simulink model "flexible_shaft_ctrl"  (R2025b)
settings: Solver=ode1be  StartTime=0.0  StopTime=simlength  FixedStep=tc  RelTol=1e-3  EnableMultiTasking=on
values from neighbouring files (symbols this model uses):
  Aled = eye(4) + Ale*ts_slow    [init.m]
  Bled = Ble*ts_slow    [init.m]
  Cle = [1 0 0 0]    [init.m]
  Dl = torque_nom/5    (= 64800)    [model1_parameters.m]    (also in model2_parameters.m = 39000; model_parameters_derivation.m = 18000)
  Dm = torque_nom/5    (= 64800)    [model1_parameters.m]    (also in model2_parameters.m = 39000; model_parameters_derivation.m = 18000)
  Dtheta = torque_nom/50    (= 6480)    [model1_parameters.m]    (also in model2_parameters.m = 3900; model_parameters_derivation.m = 18000)
  f0_min = 1/2/pi*sqrt(Ktheta*(1/Jm_max+1/Jl_max))    [model1_parameters.m]    (also in model2_parameters.m; model_parameters_derivation.m)
  Jl_model = Jl_max    [init.m]
  Jm_model = Jm_max    [init.m]
  ki = 12.5    [init.m]
  kp = 2    [init.m]
  Ksf = [0, 0, 0, 0]    [init.m]
  Lle = (lqr(Ale',Cle',Qle,Rle))'    [init.m]
  omega_nom = omega_nom_rpm/60*2*pi    (= 2.85714285714)    [model1_parameters.m]    (also in model2_parameters.m = 2.44897959184)
  omega_ref_pu = 1    [init.m]
  slope_down = 1    [init.m]
  slope_rise = 1    [init.m]
  stop = 50    [init.m]
  tc = ts_fast/2    (= 8.06451612903e-05)    [init.m]
  time_start = 0.1    [init.m]
  torque_disturbance = 0.1    [init.m]
  torque_m_pu_lim = 1.4    [init.m]
  torque_nom = 324e3    (= 324000)    [model1_parameters.m]    (also in model2_parameters.m = 195000; model_parameters_derivation.m = 180000)
  ts_fast = 1/fPWM/2    (= 0.000161290322581)    [init.m]
  ts_slow = ts_fast*SYS_TIMEBASE_FACTOR    (= 0.00129032258065)    [init.m]
  young_module_rope = 100.75e3    (= 100750)    [model1_parameters.m]    (also in model2_parameters.m; model_parameters_derivation.m = 125000)
libraries: nesl_utility x12, fl_lib x10, flexshaft_2masses_lib x2, cstblocks x1
settings Model: SimulationMode=accelerator  Creator=ltnbda  LastModifiedBy=dbagn
settings SolverCC: AlgebraicLoopSolver=TrustRegion  AutoInsertRateTranBlk=on
settings DataIOCC: LimitDataPoints=on  SaveFormat=Array  SaveOutput=off  SignalLogging=off  DSMLogging=off  SaveTime=off  ReturnWorkspaceOutputs=off
settings OptimizationCC: ReuseModelBlockBuffer=off  ExpressionDepthLimit=2147483647.0  LifeSpan=inf
settings DebuggingCC: UnderspecifiedInitializationDetection=Classic  MergeDetectMultiDrivingBlocksExec=none  SolverPrmCheckMsg=warning  UnconnectedInputMsg=warning  UnconnectedOutputMsg=warning  UnconnectedLineMsg=warning  StateNameClashWarn=warning  SFUnexpectedBacktrackingDiag=warning  SFNoUnconditionalDefaultTransitionDiag=warning  SFExecutionAtInitializationDiag=none  ArithmeticOperatorsInVariantConditions=warning
settings HardwareCC: ProdBitPerPointer=32.0  ProdBitPerSizeT=32.0  ProdBitPerPtrDiffT=32.0  ProdLargestAtomicFloat=None  ProdIntDivRoundTo=Undefined  ProdEndianess=Unspecified  ProdWordSize=32.0  ProdHWDeviceType=32-bit Generic
settings ModelReferenceCC: EnableRefExpFcnMdlSchedulingChecks=on  PropagateSignalLabelsOutOfModel=off
settings SFSimCC: SimUseLocalCustomCode=off  CustomCodeUndefinedFunction=UseInterfaceOnly
settings SFSimCC: SimCustomHeaderCode=|
  | #include "advanced_speed_control.h"
  | #include "advanced_speed_control_simulink.h"
  | #include "adv_speed_ctrl_pisf.h"
  | #include "adv_speed_ctrl_pisf_simulink.h"
  | #include "adv_speed_ctrl_pisfle.h"
  | #include "adv_speed_ctrl_pisfle_simulink.h"
settings SFSimCC: SimUserSources=|
  | "advanced_speed_control_simulink.c"
  | "advanced_speed_control.c"
  | "adv_speed_ctrl_pisf_simulink.c"
  | "adv_speed_ctrl_pisf.c"
  | "adv_speed_ctrl_pisfle_simulink.c"
  | "adv_speed_ctrl_pisfle.c"
settings SFSimCC: SimUserIncludeDirs=|
  | include
  | src
settings RTWCC: RTWUseLocalCustomCode=off  GPUComputeCapability=3.5
settings CodeAppCC: StateflowObjectComments=on
settings GRTTargetCC: TargetLangStandard=C89/C90 (ANSI)
settings ConfigComp: CovMetricSettings=dw  CovSaveCumulativeToWorkspaceVar=on  CovSaveSingleToWorkspaceVar=on  CovExternalEMLEnable=off

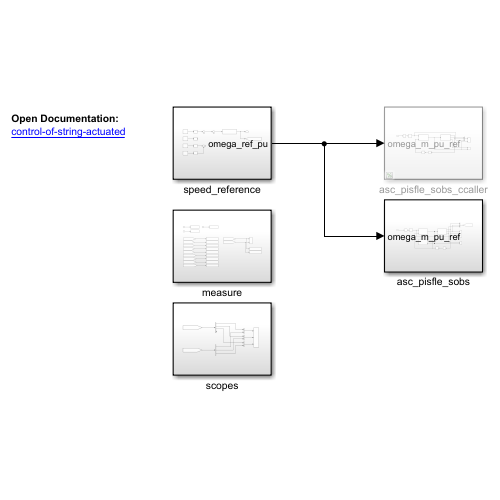
[thumbnail: Simulink's stored preview of the top-level diagram]
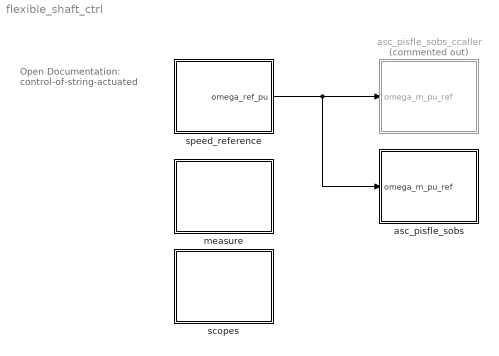
== system flexible_shaft_ctrl ==
  note: Open Documentation:
      | control-of-string-actuated
  asc_pisfle_sobs : Subsystem
  asc_pisfle_sobs_ccaller : Subsystem  Commented=on
  measure : Subsystem
  scopes : Subsystem
  speed_reference : Subsystem
  wires:
  speed_reference/1(omega_ref_pu) -> asc_pisfle_sobs_ccaller/1(omega_m_pu_ref), asc_pisfle_sobs/1(omega_m_pu_ref)

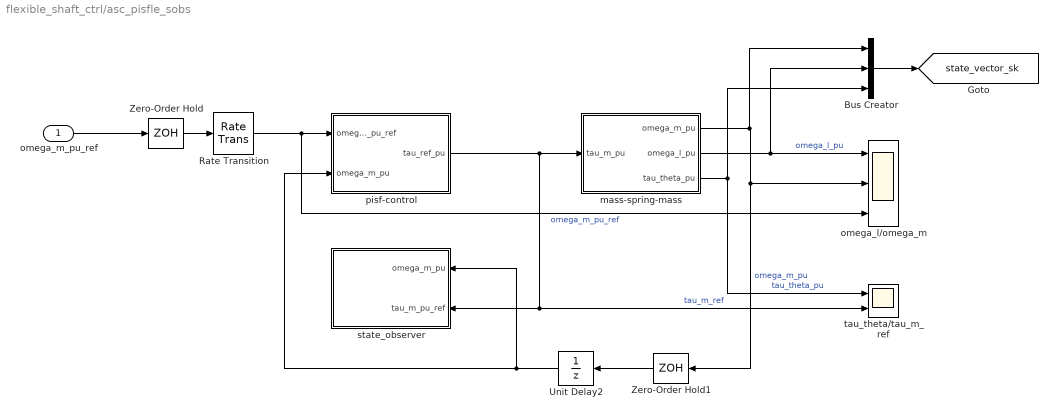
== system flexible_shaft_ctrl/asc_pisfle_sobs ==
  omega_m_pu_ref : Inport
  Bus Creator : BusCreator  Inputs=3
  Rate Transition : RateTransition  OutPortSampleTime=ts_slow
  Unit Delay2 : UnitDelay  SampleTime=ts_slow  HasFrameUpgradeWarning=on
  Zero-Order Hold : ZeroOrderHold  SampleTime=ts_slow
  Zero-Order Hold1 : ZeroOrderHold  SampleTime=ts_slow
  mass-spring-mass : Subsystem
  omega_l/omega_m : Scope  NumInputPorts=3
      settings: ActiveDisplayYMinimum=-0.17271134973649729  ActiveDisplayYMaximum=1.5544021476284759
  pisf-control : Subsystem
  state_observer : Subsystem
  tau_theta/tau_m_ref : Scope  NumInputPorts=2
      settings: ActiveDisplayYMinimum=-1.2903878055625353  ActiveDisplayYMaximum=1.6989319783958372
  tag scope: state_vector_sk=global
  wires:
  Unit Delay2/1 -> state_observer/1(omega_m_pu), pisf-control/2(omega_m_pu)
  mass-spring-mass/2(omega_l_pu) -> Bus Creator/2, omega_l/omega_m/1  "omega_l_pu"
  Zero-Order Hold1/1 -> Unit Delay2/1
  mass-spring-mass/1(omega_m_pu) -> Bus Creator/1, Zero-Order Hold1/1, omega_l/omega_m/2  "omega_m_pu"
  mass-spring-mass/3(tau_theta_pu) -> Bus Creator/3, tau_theta/tau_m_ref/1  "tau_theta_pu"
  omega_m_pu_ref/1 -> Zero-Order Hold/1
  Rate Transition/1 -> pisf-control/1(omega_m_pu_ref), omega_l/omega_m/3  "omega_m_pu_ref"
  pisf-control/1(tau_ref_pu) -> state_observer/2(tau_m_pu_ref), tau_theta/tau_m_ref/2, mass-spring-mass/1(tau_m_pu)  "tau_m_ref"
  Zero-Order Hold/1 -> Rate Transition/1
  Bus Creator/1 -> [state_vector_sk]

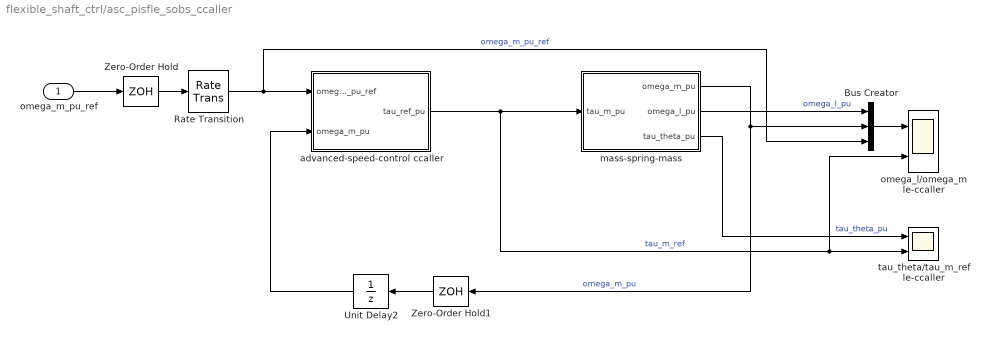
== system flexible_shaft_ctrl/asc_pisfle_sobs_ccaller ==
  omega_m_pu_ref : Inport
  Bus Creator : BusCreator  Inputs=3
  Rate Transition : RateTransition  OutPortSampleTime=ts_slow
  Unit Delay2 : UnitDelay  SampleTime=ts_slow  HasFrameUpgradeWarning=on
  Zero-Order Hold : ZeroOrderHold  SampleTime=ts_slow
  Zero-Order Hold1 : ZeroOrderHold  SampleTime=ts_slow
  advanced-speed-control ccaller : Subsystem
  mass-spring-mass : Subsystem
  omega_l/omega_m le-ccaller : Scope  NumInputPorts=2
      settings: SampleTime=ts_slow  ActiveDisplayYMinimum=-0.2317  ActiveDisplayYMaximum=2.0853
  tau_theta/tau_m_ref le-ccaller : Scope  NumInputPorts=2
      settings: SampleTime=tc  ActiveDisplayYMinimum=-0.175  ActiveDisplayYMaximum=1.575
  wires:
  Unit Delay2/1 -> advanced-speed-control ccaller/2(omega_m_pu)
  mass-spring-mass/2(omega_l_pu) -> Bus Creator/1  "omega_l_pu"
  Zero-Order Hold1/1 -> Unit Delay2/1
  mass-spring-mass/1(omega_m_pu) -> Bus Creator/2, Zero-Order Hold1/1  "omega_m_pu"
  mass-spring-mass/3(tau_theta_pu) -> tau_theta/tau_m_ref le-ccaller/1  "tau_theta_pu"
  omega_m_pu_ref/1 -> Zero-Order Hold/1
  Zero-Order Hold/1 -> Rate Transition/1
  advanced-speed-control ccaller/1(tau_ref_pu) -> omega_l/omega_m le-ccaller/2, tau_theta/tau_m_ref le-ccaller/2, mass-spring-mass/1(tau_m_pu)  "tau_m_ref"
  Bus Creator/1 -> omega_l/omega_m le-ccaller/1
  Rate Transition/1 -> Bus Creator/3, advanced-speed-control ccaller/1(omega_m_pu_ref)  "omega_m_pu_ref"

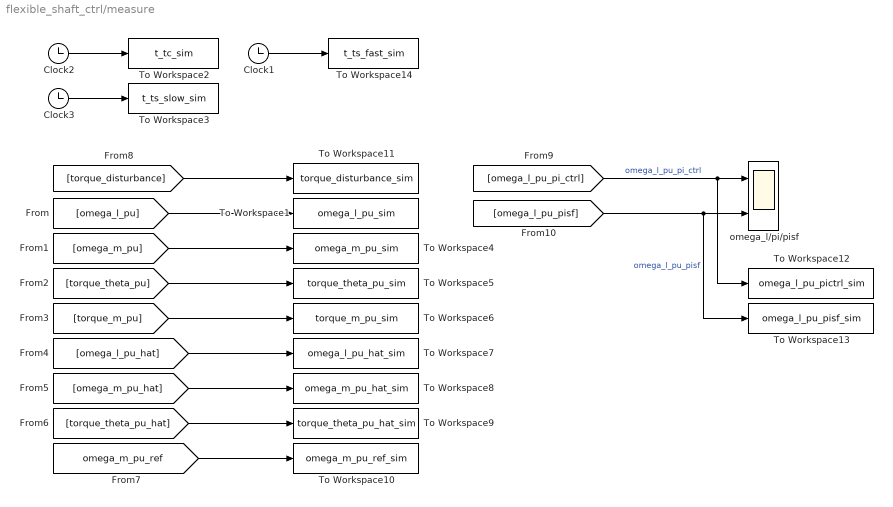
== system flexible_shaft_ctrl/measure ==
  Clock1 : Clock
  Clock2 : Clock
  Clock3 : Clock
  To Workspace1 : ToWorkspace  VariableName=omega_l_pu_sim  SampleTime=tc
      settings: MaxDataPoints=Nc
  To Workspace10 : ToWorkspace  VariableName=omega_m_pu_ref_sim  SampleTime=tc
      settings: MaxDataPoints=Nc
  To Workspace11 : ToWorkspace  VariableName=torque_disturbance_sim  SampleTime=tc
      settings: MaxDataPoints=Nc
  To Workspace12 : ToWorkspace  VariableName=omega_l_pu_pictrl_sim  SampleTime=tc
      settings: MaxDataPoints=Nc
  To Workspace13 : ToWorkspace  VariableName=omega_l_pu_pisf_sim  SampleTime=tc
      settings: MaxDataPoints=Nc
  To Workspace14 : ToWorkspace  VariableName=t_ts_fast_sim  SampleTime=ts_fast
      settings: MaxDataPoints=Ns_fast
  To Workspace2 : ToWorkspace  VariableName=t_tc_sim  SampleTime=tc
      settings: MaxDataPoints=Nc
  To Workspace3 : ToWorkspace  VariableName=t_ts_slow_sim  SampleTime=ts_slow
      settings: MaxDataPoints=Ns_slow
  To Workspace4 : ToWorkspace  VariableName=omega_m_pu_sim  SampleTime=tc
      settings: MaxDataPoints=Nc
  To Workspace5 : ToWorkspace  VariableName=torque_theta_pu_sim  SampleTime=tc
      settings: MaxDataPoints=Nc
  To Workspace6 : ToWorkspace  VariableName=torque_m_pu_sim  SampleTime=tc
      settings: MaxDataPoints=Nc
  To Workspace7 : ToWorkspace  VariableName=omega_l_pu_hat_sim  SampleTime=tc
      settings: MaxDataPoints=Nc
  To Workspace8 : ToWorkspace  VariableName=omega_m_pu_hat_sim  SampleTime=tc
      settings: MaxDataPoints=Nc
  To Workspace9 : ToWorkspace  VariableName=torque_theta_pu_hat_sim  SampleTime=tc
      settings: MaxDataPoints=Nc
  omega_l/pi/pisf : Scope  NumInputPorts=2
      settings: SampleTime=tc  ActiveDisplayYMinimum=-0.18711  ActiveDisplayYMaximum=1.68397
  wires:
  Clock2/1 -> To Workspace2/1
  Clock3/1 -> To Workspace3/1
  [omega_l_pu] -> To Workspace1/1
  [omega_m_pu] -> To Workspace4/1
  [torque_theta_pu] -> To Workspace5/1
  [torque_m_pu] -> To Workspace6/1
  [omega_l_pu_hat] -> To Workspace7/1
  [omega_m_pu_hat] -> To Workspace8/1
  [torque_theta_pu_hat] -> To Workspace9/1
  [omega_m_pu_ref] -> To Workspace10/1
  [torque_disturbance] -> To Workspace11/1
  [omega_l_pu_pisf] -> To Workspace13/1, omega_l/pi/pisf/2  "omega_l_pu_pisf"
  [omega_l_pu_pi_ctrl] -> To Workspace12/1, omega_l/pi/pisf/1  "omega_l_pu_pi_ctrl"
  Clock1/1 -> To Workspace14/1

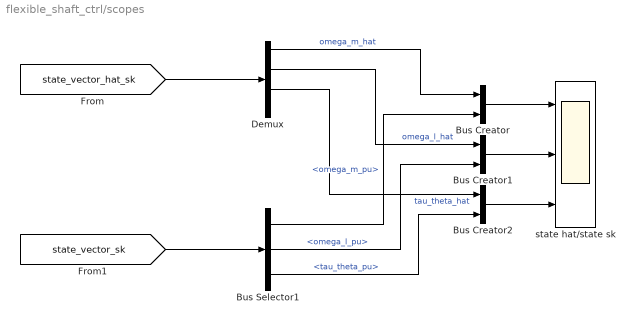
== system flexible_shaft_ctrl/scopes ==
  Bus Creator : BusCreator  Inputs=2
  Bus Creator1 : BusCreator  Inputs=2
  Bus Creator2 : BusCreator  Inputs=2
  Bus Selector1 : BusSelector  OutputSignals=omega_m_pu,omega_l_pu,tau_theta_pu
  Demux : Demux
  state hat/state sk : Scope  NumInputPorts=3
      settings: ActiveDisplayString=3  ActiveDisplayYMinimum=-0.14809096846427292  ActiveDisplayYMaximum=1.3328187161784566  DataLoggingVariableName=ScopeData2
  wires:
  [state_vector_hat_sk] -> Demux/1
  [state_vector_sk] -> Bus Selector1/1
  Bus Selector1/1 -> Bus Creator/2  "<omega_m_pu>"
  Bus Selector1/2 -> Bus Creator1/2  "<omega_l_pu>"
  Bus Selector1/3 -> Bus Creator2/2  "<tau_theta_pu>"
  Bus Creator/1 -> state hat/state sk/1
  Demux/1 -> Bus Creator/1  "omega_m_hat"
  Bus Creator2/1 -> state hat/state sk/3
  Bus Creator1/1 -> state hat/state sk/2
  Demux/2 -> Bus Creator1/1  "omega_l_hat"
  Demux/3 -> Bus Creator2/1  "tau_theta_hat"

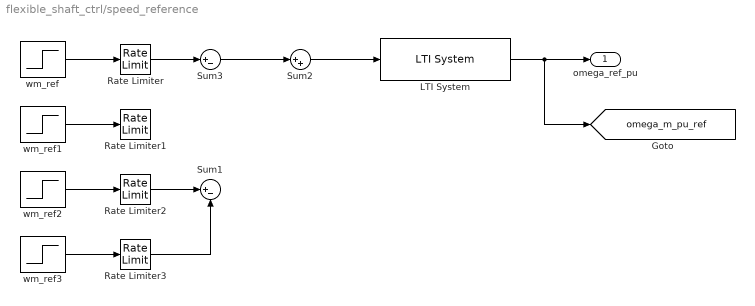
== system flexible_shaft_ctrl/speed_reference ==
  LTI System : cstblocks/LTI System  sys=lowpassfilter_snd_d  IC=[]  PadeOrder=0
  Rate Limiter : RateLimiter  RisingSlewLimit=omega_ref_pu*slope_rise  FallingSlewLimit=-omega_ref_pu*slope_rise
  Rate Limiter1 : RateLimiter  RisingSlewLimit=omega_ref_pu*slope_down  FallingSlewLimit=-omega_ref_pu*slope_down
  Rate Limiter2 : RateLimiter  RisingSlewLimit=omega_ref_pu*slope_rise  FallingSlewLimit=-omega_ref_pu*slope_rise
  Rate Limiter3 : RateLimiter  RisingSlewLimit=omega_ref_pu*slope_down  FallingSlewLimit=-omega_ref_pu*slope_down
  Sum1 : Sum  Inputs=|+-
  Sum2 : Sum  Inputs=|++
  Sum3 : Sum  Inputs=|+-
  wm_ref : Step  Time=time_start  After=omega_ref_pu  SampleTime=0
  wm_ref1 : Step  Time=time_start+stop  After=2*omega_ref_pu  SampleTime=0
  wm_ref2 : Step  Time=time_start+2*stop  After=omega_ref_pu  SampleTime=0
  wm_ref3 : Step  Time=time_start+3*stop  After=omega_ref_pu  SampleTime=0
  omega_ref_pu : Outport  VectorParamsAs1DForOutWhenUnconnected=off
  tag scope: omega_m_pu_ref=global
  wires:
  wm_ref1/1 -> Rate Limiter1/1
  wm_ref/1 -> Rate Limiter/1
  Sum2/1 -> LTI System/1
  Rate Limiter/1 -> Sum3/1
  LTI System/1 -> [omega_m_pu_ref], omega_ref_pu/1
  wm_ref3/1 -> Rate Limiter3/1
  wm_ref2/1 -> Rate Limiter2/1
  Rate Limiter2/1 -> Sum1/1
  Rate Limiter3/1 -> Sum1/2
  Sum3/1 -> Sum2/1

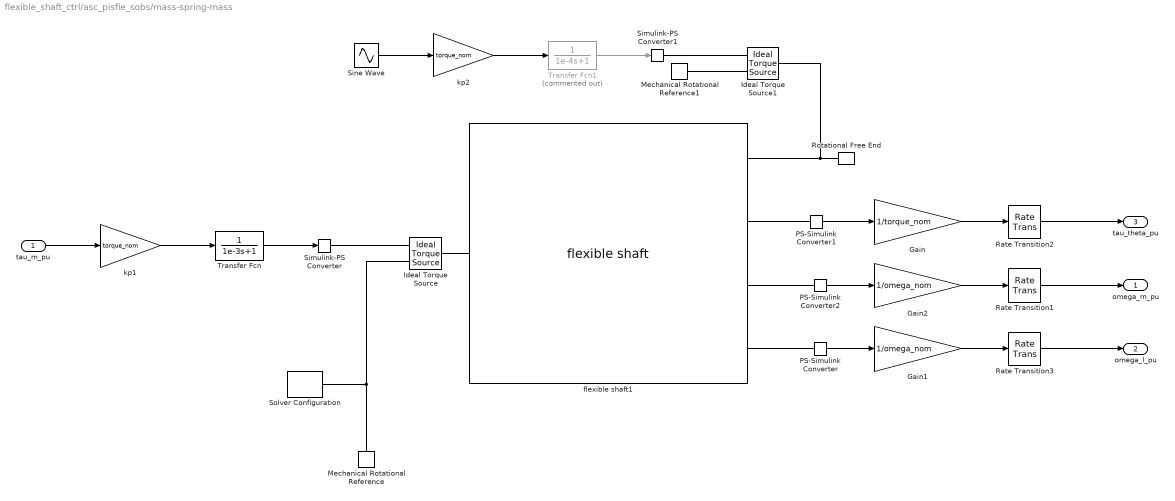
== system flexible_shaft_ctrl/asc_pisfle_sobs/mass-spring-mass ==
  tau_m_pu : Inport
  Gain : Gain  Gain=1/torque_nom
  Gain1 : Gain  Gain=1/omega_nom
  Gain2 : Gain  Gain=1/omega_nom
  Ideal Torque Source : fl_lib/Mechanical/Mechanical Sources/Ideal Torque Source
  Ideal Torque Source1 : fl_lib/Mechanical/Mechanical Sources/Ideal Torque Source
  Mechanical Rotational Reference : fl_lib/Mechanical/Rotational Elements/Mechanical Rotational Reference
  Mechanical Rotational Reference1 : fl_lib/Mechanical/Rotational Elements/Mechanical Rotational Reference
  PS-Simulink Converter : nesl_utility/PS-Simulink Converter  PhysicalDomain=network_engine_domain  SubClassName=ps_output  LeftPortType=input  RightPortType=output  PseudoPeriodic=off  Frequencies=[]  VectorFormat=1-D array  Unit=rad/s  AffineConversion=off
  PS-Simulink Converter1 : nesl_utility/PS-Simulink Converter  PhysicalDomain=network_engine_domain  SubClassName=ps_output  LeftPortType=input  RightPortType=output  PseudoPeriodic=off  Frequencies=[]  VectorFormat=1-D array  Unit=N*m  AffineConversion=off
  PS-Simulink Converter2 : nesl_utility/PS-Simulink Converter  PhysicalDomain=network_engine_domain  SubClassName=ps_output  LeftPortType=input  RightPortType=output  PseudoPeriodic=off  Frequencies=[]  VectorFormat=1-D array  Unit=rad/s  AffineConversion=off
  Rate Transition1 : RateTransition  OutPortSampleTime=ts_slow
  Rate Transition2 : RateTransition  OutPortSampleTime=ts_slow
  Rate Transition3 : RateTransition  OutPortSampleTime=ts_slow
  Rotational Free End : fl_lib/Mechanical/Rotational Elements/Rotational Free End  w_specify=off  w_priority=None  w=0 rad/s  w_nominal_specify=off  w_nominal_value=1  w_nominal_unit=rad/s
  Simulink-PS Converter : nesl_utility/Simulink-PS Converter  PhysicalDomain=network_engine_domain  SubClassName=ps_input  LeftPortType=input  RightPortType=output  PseudoPeriodic=off  Frequencies=[]  NoiseDistribution=none  NoiseParameters=[]  Unit=N*m  AffineConversion=off  FilteringAndDerivatives=provide  SimscapeFilterOrder=1  InputFilterTimeConstant=0.001  UdotUserProvided=0
  Simulink-PS Converter1 : nesl_utility/Simulink-PS Converter  PhysicalDomain=network_engine_domain  SubClassName=ps_input  LeftPortType=input  RightPortType=output  PseudoPeriodic=off  Frequencies=[]  NoiseDistribution=none  NoiseParameters=[]  Unit=N*m  AffineConversion=off  FilteringAndDerivatives=provide  SimscapeFilterOrder=1  InputFilterTimeConstant=0.001  UdotUserProvided=0
  Sine Wave : Sin  Amplitude=torque_disturbance  Frequency=f0_min*2*pi  SampleTime=0
  Solver Configuration : nesl_utility/Solver Configuration  PhysicalDomain=network_engine_domain  SubClassName=solver  LeftPortType=input  RightPortType=generic  Tones=[]  Harmonics=[]  SimulateNoise=off  Profile=off  UseLocalSampling=off  EnableSwitchedLinearOptims=on  FrequencyDomain=off  UseCCode=off  RelTol=0.001  AbsTol=0.001  MinStep=1e-09  ToWorkspace=off  RevertToSquareIcSolve=off  NumHomotopyIterations=100  PhasorMode=off  PhasorModeNumHarmonics=1  ConsistencySolver=NEWTON_XTOL_AFTER_FTOL  IndexReductionMethod=DerivativeReplacement  DoDC=off  ResidualTolerance=1e-09  ConsistencyTolSource=GLOBAL  ConsistencyAbsTol=0.001  ConsistencyRelTol=0.001  ConsistencyTolFactor=0.001  UseLocalSolver=on  LocalSolverChoice=NE_BACKWARD_EULER_ADVANCER  ResolveIndetEquations=on  FunctionEvalNumThread=1  LocalSolverSampleTime=tc  DoFixedCost=on  MaxNonlinIter=3  MaxModeIter=2  ComputeImpulses=off  ImpulseIterations=2  LinearAlgebra=auto  LinearAlgebraNumThread=0  EquationFormulation=NE_TIME_EF  DelaysMemoryBudget=1024  AutomaticFiltering=on  FilteringTimeConstant=0.001  PartitionStorageMethod=AS_NEEDED  PartitionMemoryBudget=1024  PartitionMethod=ROBUST  MultibodyUseLocalSolver=off  MultibodyLocalSolverChoice=ODE1  MultibodyLocalSolverSampleTime=0.001
  Transfer Fcn : TransferFcn  Denominator=[1e-3 1]
  Transfer Fcn1 : TransferFcn  Commented=on  Denominator=[1e-4 1]
  flexible shaft1 : flexshaft_2masses_lib/flexible shaft  b1=Dm N*m*s/rad  J1=Jm_model kg*m^2  b2=Dl N*m*s/rad  J2=Jl_model kg*m^2  b_theta=Dtheta N*m*s/rad  k_theta=Ktheta_model N*m/rad  w_1_specify=off  w_1_priority=None  w_1=0 rad/s  w_1_nominal_specify=off  w_1_nominal_value=1  w_1_nominal_unit=rad/s  w_2_specify=off  w_2_priority=None  w_2=0 rad/s  w_2_nominal_specify=off  w_2_nominal_value=1  w_2_nominal_unit=rad/s  t_1_specify=off  t_1_priority=None  t_1=0 N*m  t_1_nominal_specify=off  t_1_nominal_value=1  t_1_nominal_unit=N*m  t_2_specify=off  t_2_priority=None  t_2=0 N*m  t_2_nominal_specify=off  t_2_nominal_value=1  t_2_nominal_unit=N*m  t_theta_specify=off  t_theta_priority=None  t_theta=0 N*m  t_theta_nominal_specify=off  t_theta_nominal_value=1  t_theta_nominal_unit=N*m
      settings: InternalSimscapePortConfiguration="{\"Bottom\":[],\"Left\":[{\"id\":\"S1\",\"label\":\"S1\",\"type\":\"foundation.mechanical.rotational.rotational\"}],\"Right\":[{\"id\":\"S2\",\"label\":\"S2\",\"type\":\"foundation.mechanical.rotational.rotational\"},{\"id\":\"tau_theta\",\"label\":\"tau_theta\",\"type\":\"output\"},{\"id\":\"w1\",\"label\":\"w1\",\"type\":\"output\"},{\"id\":\"w2\",\"label\":\"w2\",\"type\":\"output\"}],\"Top\":[]}"
  kp1 : Gain  Gain=torque_nom  SaturateOnIntegerOverflow=on  OutDataTypeStr=Inherit: Same as input  ParamDataTypeStr=Inherit: Same as input
  kp2 : Gain  Gain=torque_nom  SaturateOnIntegerOverflow=on  OutDataTypeStr=Inherit: Same as input  ParamDataTypeStr=Inherit: Same as input
  omega_m_pu : Outport
  omega_l_pu : Outport  Port=2
  tau_theta_pu : Outport  Port=3
  wires:
  Sine Wave/1 -> kp2/1
  kp2/1 -> Transfer Fcn1/1
  Transfer Fcn1/1 -> Simulink-PS Converter1/1
  tau_m_pu/1 -> kp1/1
  PS-Simulink Converter2/1 -> Gain2/1
  PS-Simulink Converter/1 -> Gain1/1
  PS-Simulink Converter1/1 -> Gain/1
  Gain/1 -> Rate Transition2/1
  Gain1/1 -> Rate Transition3/1
  Gain2/1 -> Rate Transition1/1
  Transfer Fcn/1 -> Simulink-PS Converter/1
  kp1/1 -> Transfer Fcn/1
  Rate Transition2/1 -> tau_theta_pu/1
  Rate Transition1/1 -> omega_m_pu/1
  Rate Transition3/1 -> omega_l_pu/1
  connections:
  Simulink-PS Converter1/RConn1 -- Ideal Torque Source1/RConn1
  Mechanical Rotational Reference1/LConn1 -- Ideal Torque Source1/RConn2
  Ideal Torque Source1/LConn1 -- Rotational Free End/LConn1 -- flexible shaft1/RConn1
  Ideal Torque Source/RConn1 -- Simulink-PS Converter/RConn1
  flexible shaft1/LConn1 -- Ideal Torque Source/LConn1
  Mechanical Rotational Reference/LConn1 -- Solver Configuration/RConn1 -- Ideal Torque Source/RConn2
  flexible shaft1/RConn4 -- PS-Simulink Converter/LConn1
  flexible shaft1/RConn2 -- PS-Simulink Converter1/LConn1
  flexible shaft1/RConn3 -- PS-Simulink Converter2/LConn1

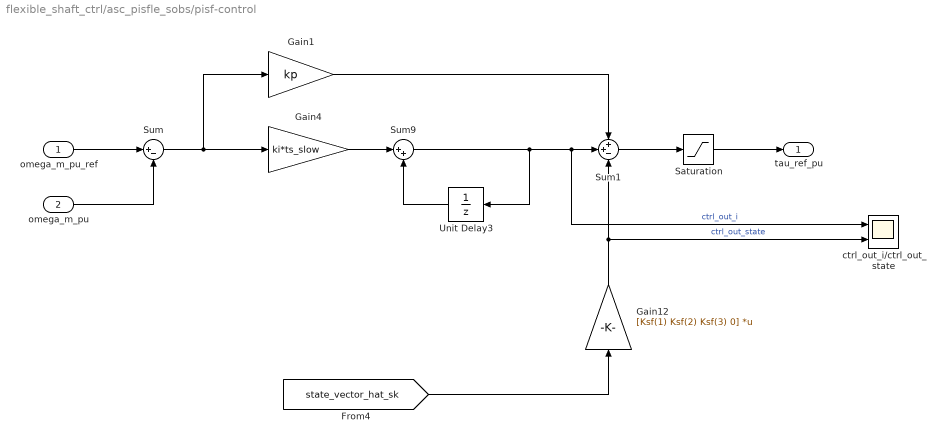
== system flexible_shaft_ctrl/asc_pisfle_sobs/pisf-control ==
  omega_m_pu_ref : Inport
  omega_m_pu : Inport  Port=2
  Gain1 : Gain  Gain=kp
  Gain12 : Gain  Gain=[Ksf(1) Ksf(2) Ksf(3) 0]  Multiplication=Matrix(K*u)
  Gain4 : Gain  Gain=ki*ts_slow
  Saturation : Saturate  UpperLimit=torque_m_pu_lim  LowerLimit=-torque_m_pu_lim
  Sum : Sum  Inputs=|+-
  Sum1 : Sum  Inputs=++-
  Sum9 : Sum  Inputs=|++
  Unit Delay3 : UnitDelay  SampleTime=ts_slow  HasFrameUpgradeWarning=on
  ctrl_out_i/ctrl_out_state : Scope  NumInputPorts=2
      settings: SampleTime=tc  ActiveDisplayYMinimum=-840.27141275796646  ActiveDisplayYMaximum=7562.4427148217
  tau_ref_pu : Outport  VectorParamsAs1DForOutWhenUnconnected=off
  wires:
  omega_m_pu_ref/1 -> Sum/1
  omega_m_pu/1 -> Sum/2
  Sum/1 -> Gain1/1, Gain4/1
  Gain4/1 -> Sum9/1
  [state_vector_hat_sk] -> Gain12/1
  Sum1/1 -> Saturation/1
  Sum9/1 -> ctrl_out_i/ctrl_out_state/1, Sum1/2, Unit Delay3/1  "ctrl_out_i"
  Gain1/1 -> Sum1/1
  Unit Delay3/1 -> Sum9/2
  Gain12/1 -> Sum1/3, ctrl_out_i/ctrl_out_state/2  "ctrl_out_state"
  Saturation/1 -> tau_ref_pu/1

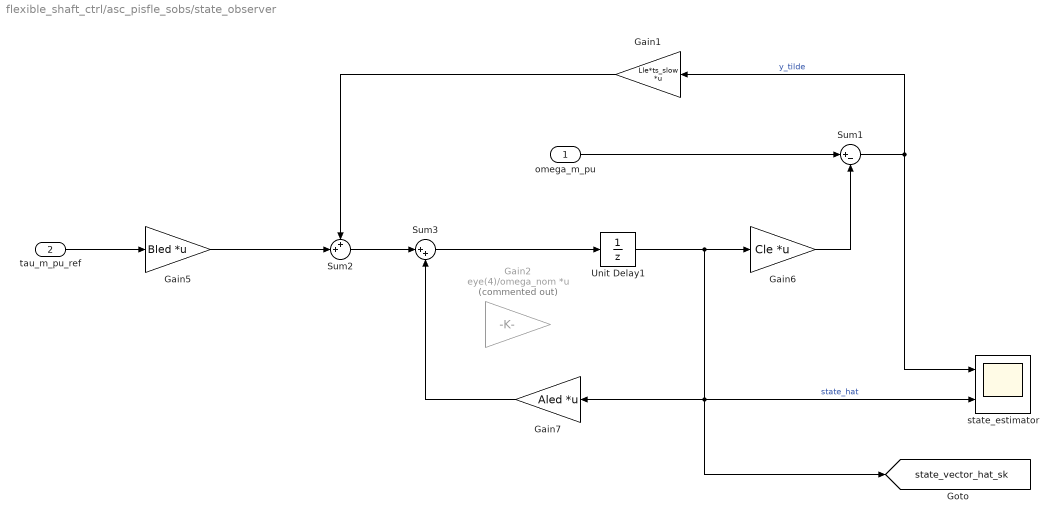
== system flexible_shaft_ctrl/asc_pisfle_sobs/state_observer ==
  omega_m_pu : Inport
  tau_m_pu_ref : Inport  Port=2
  Gain1 : Gain  Gain=Lle*ts_slow  Multiplication=Matrix(K*u)
  Gain2 : Gain  Commented=on  Gain=eye(4)/omega_nom  Multiplication=Matrix(K*u)
  Gain5 : Gain  Gain=Bled  Multiplication=Matrix(K*u)
  Gain6 : Gain  Gain=Cle  Multiplication=Matrix(K*u)
  Gain7 : Gain  Gain=Aled  Multiplication=Matrix(K*u)
  Sum1 : Sum  Inputs=|+-
  Sum2 : Sum  Inputs=++|
  Sum3 : Sum  Inputs=|++
  Unit Delay1 : UnitDelay  InitialCondition=[0 0 0 0]  SampleTime=ts_slow  HasFrameUpgradeWarning=on
  state_estimator : Scope  NumInputPorts=2
      settings: SampleTime=tc  ActiveDisplayYMinimum=-0.10921755337632549  ActiveDisplayYMaximum=0.028869122548924514
  tag scope: state_vector_hat_sk=global
  wires:
  omega_m_pu/1 -> Sum1/1
  Sum1/1 -> Gain1/1, state_estimator/1  "y_tilde"
  tau_m_pu_ref/1 -> Gain5/1
  Gain6/1 -> Sum1/2
  Sum2/1 -> Sum3/1
  Gain5/1 -> Sum2/2
  Gain7/1 -> Sum3/2
  Unit Delay1/1 -> Gain6/1, [state_vector_hat_sk], state_estimator/2, Gain7/1  "state_hat"
  Gain1/1 -> Sum2/1
  Sum3/1 -> Unit Delay1/1

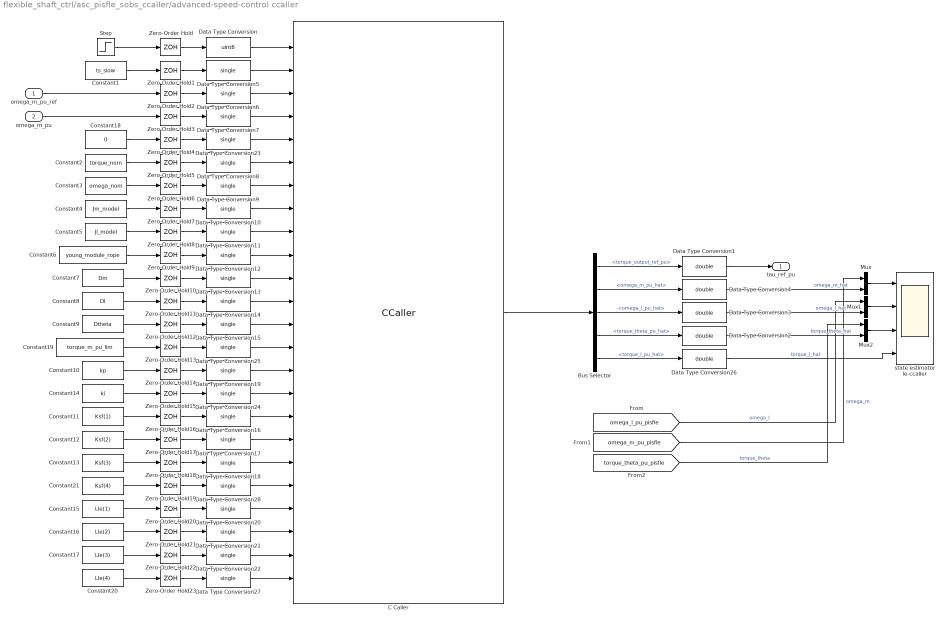
== system flexible_shaft_ctrl/asc_pisfle_sobs_ccaller/advanced-speed-control ccaller ==
  omega_m_pu_ref : Inport
  omega_m_pu : Inport  Port=2
  Bus Selector : BusSelector  OutputSignals=torque_output_ref_pu,omega_m_pu_hat,omega_l_pu_hat,torque_theta_pu_hat,torque_l_pu_hat
  C Caller : CCaller  FunctionName=adv_speed_ctrl_pisfle_process_simulink  PortSpecificationStruct="%)30     .    6\"L   8    (     @         %    \"    !D    !     0         %  0 \"0    $    _    07)G3F%M90  4&]R=$YA;64 4V-O<&4     26YD97@     5'EP90      4VEZ90      27-';&]B86P   X    P    !@    @    $          4    (     0    ,    !         !   P!O=70 #@   #     &    \"     0         !0    @    !     P    $         $  # &]U=  .    .     8    (    !          %    \"     $    &     0         0  ...(+14588 chars)"  SampleTime=ts_slow
  Constant1 : Constant  Value=ts_slow
  Constant10 : Constant  Value=kp
  Constant11 : Constant  Value=Ksf(1)
  Constant12 : Constant  Value=Ksf(2)
  Constant13 : Constant  Value=Ksf(3)
  Constant14 : Constant  Value=ki
  Constant15 : Constant  Value=Lle(1)
  Constant16 : Constant  Value=Lle(2)
  Constant17 : Constant  Value=Lle(3)
  Constant18 : Constant  Value=0
  Constant19 : Constant  Value=torque_m_pu_lim
  Constant2 : Constant  Value=torque_nom
  Constant20 : Constant  Value=Lle(4)
  Constant21 : Constant  Value=Ksf(4)
  Constant3 : Constant  Value=omega_nom
  Constant4 : Constant  Value=Jm_model
  Constant5 : Constant  Value=Jl_model
  Constant6 : Constant  Value=young_module_rope
  Constant7 : Constant  Value=Dm
  Constant8 : Constant  Value=Dl
  Constant9 : Constant  Value=Dtheta
  Data Type Conversion : DataTypeConversion  OutDataTypeStr=uint8  SaturateOnIntegerOverflow=off  RndMeth=Floor
  Data Type Conversion{1..4,26} (5 alike) : DataTypeConversion  OutDataTypeStr=double  SaturateOnIntegerOverflow=off  RndMeth=Floor
  Data Type Conversion{5..25,27..28} (23 alike) : DataTypeConversion  OutDataTypeStr=single  SaturateOnIntegerOverflow=off  RndMeth=Floor
  Mux : Mux  Inputs=2
  Mux1 : Mux  Inputs=2
  Mux2 : Mux  Inputs=2
  Step : Step  Time=0.1  Before=1  After=0  SampleTime=0
  Zero-Order Hold{,1..23} (24 alike) : ZeroOrderHold  SampleTime=ts_slow
  state estimator le-ccaller : Scope  NumInputPorts=4
      settings: SampleTime=ts_slow  ActiveDisplayYMinimum=-0.19605  ActiveDisplayYMaximum=1.76442
  tau_ref_pu : Outport  VectorParamsAs1DForOutWhenUnconnected=off
  wires:
  Data Type Conversion28/1 -> C Caller/20
  Constant21/1 -> Zero-Order Hold19/1
  Zero-Order Hold19/1 -> Data Type Conversion28/1
  Data Type Conversion27/1 -> C Caller/24
  Constant20/1 -> Zero-Order Hold23/1
  Zero-Order Hold23/1 -> Data Type Conversion27/1
  Data Type Conversion22/1 -> C Caller/23
  Data Type Conversion21/1 -> C Caller/22
  Data Type Conversion20/1 -> C Caller/21
  Bus Selector/1 -> Data Type Conversion1/1  "<torque_output_ref_pu>"
  Data Type Conversion26/1 -> state estimator le-ccaller/4  "torque_l_hat"
  Bus Selector/5 -> Data Type Conversion26/1  "<torque_l_pu_hat>"
  Bus Selector/4 -> Data Type Conversion2/1  "<torque_theta_pu_hat>"
  Bus Selector/3 -> Data Type Conversion3/1  "<omega_l_pu_hat>"
  Bus Selector/2 -> Data Type Conversion4/1  "<omega_m_pu_hat>"
  Zero-Order Hold13/1 -> Data Type Conversion25/1
  Constant19/1 -> Zero-Order Hold13/1
  Data Type Conversion25/1 -> C Caller/14
  Data Type Conversion18/1 -> C Caller/19
  Data Type Conversion17/1 -> C Caller/18
  Data Type Conversion16/1 -> C Caller/17
  Data Type Conversion24/1 -> C Caller/16
  Data Type Conversion19/1 -> C Caller/15
  Constant10/1 -> Zero-Order Hold14/1
  Zero-Order Hold14/1 -> Data Type Conversion19/1
  Zero-Order Hold15/1 -> Data Type Conversion24/1
  Constant14/1 -> Zero-Order Hold15/1
  Data Type Conversion3/1 -> Mux1/2  "omega_l_hat"
  Data Type Conversion4/1 -> Mux/2  "omega_m_hat"
  Data Type Conversion2/1 -> Mux2/2  "torque_theta_hat"
  Data Type Conversion1/1 -> tau_ref_pu/1
  Data Type Conversion23/1 -> C Caller/5
  Constant18/1 -> Zero-Order Hold4/1
  Zero-Order Hold4/1 -> Data Type Conversion23/1
  Zero-Order Hold20/1 -> Data Type Conversion20/1
  Constant15/1 -> Zero-Order Hold20/1
  Constant16/1 -> Zero-Order Hold21/1
  Zero-Order Hold21/1 -> Data Type Conversion21/1
  Zero-Order Hold22/1 -> Data Type Conversion22/1
  Constant17/1 -> Zero-Order Hold22/1
  Zero-Order Hold18/1 -> Data Type Conversion18/1
  Constant13/1 -> Zero-Order Hold18/1
  Constant12/1 -> Zero-Order Hold17/1
  Zero-Order Hold17/1 -> Data Type Conversion17/1
  Zero-Order Hold16/1 -> Data Type Conversion16/1
  Constant11/1 -> Zero-Order Hold16/1
  Data Type Conversion15/1 -> C Caller/13
  Constant9/1 -> Zero-Order Hold12/1
  Zero-Order Hold12/1 -> Data Type Conversion15/1
  Data Type Conversion14/1 -> C Caller/12
  Zero-Order Hold11/1 -> Data Type Conversion14/1
  Constant8/1 -> Zero-Order Hold11/1
  Data Type Conversion13/1 -> C Caller/11
  Constant7/1 -> Zero-Order Hold10/1
  Zero-Order Hold10/1 -> Data Type Conversion13/1
  Data Type Conversion12/1 -> C Caller/10
  Zero-Order Hold9/1 -> Data Type Conversion12/1
  Constant6/1 -> Zero-Order Hold9/1
  Data Type Conversion11/1 -> C Caller/9
  Constant5/1 -> Zero-Order Hold8/1
  Zero-Order Hold8/1 -> Data Type Conversion11/1
  Data Type Conversion10/1 -> C Caller/8
  Zero-Order Hold7/1 -> Data Type Conversion10/1
  Constant4/1 -> Zero-Order Hold7/1
  Data Type Conversion9/1 -> C Caller/7
  Constant3/1 -> Zero-Order Hold6/1
  Zero-Order Hold6/1 -> Data Type Conversion9/1
  Data Type Conversion8/1 -> C Caller/6
  Zero-Order Hold5/1 -> Data Type Conversion8/1
  Constant2/1 -> Zero-Order Hold5/1
  Zero-Order Hold3/1 -> Data Type Conversion7/1
  omega_m_pu/1 -> Zero-Order Hold3/1
  Data Type Conversion7/1 -> C Caller/4
  omega_m_pu_ref/1 -> Zero-Order Hold2/1
  Data Type Conversion6/1 -> C Caller/3
  Zero-Order Hold2/1 -> Data Type Conversion6/1
  Data Type Conversion5/1 -> C Caller/2
  Constant1/1 -> Zero-Order Hold1/1
  Zero-Order Hold1/1 -> Data Type Conversion5/1
  Data Type Conversion/1 -> C Caller/1
  Zero-Order Hold/1 -> Data Type Conversion/1
  Step/1 -> Zero-Order Hold/1
  C Caller/1 -> Bus Selector/1
  [omega_l_pu_pisfle] -> Mux1/1  "omega_l"
  [omega_m_pu_pisfle] -> Mux/1  "omega_m"
  [torque_theta_pu_pisfle] -> Mux2/1  "torque_theta"
  Mux2/1 -> state estimator le-ccaller/3
  Mux1/1 -> state estimator le-ccaller/2
  Mux/1 -> state estimator le-ccaller/1

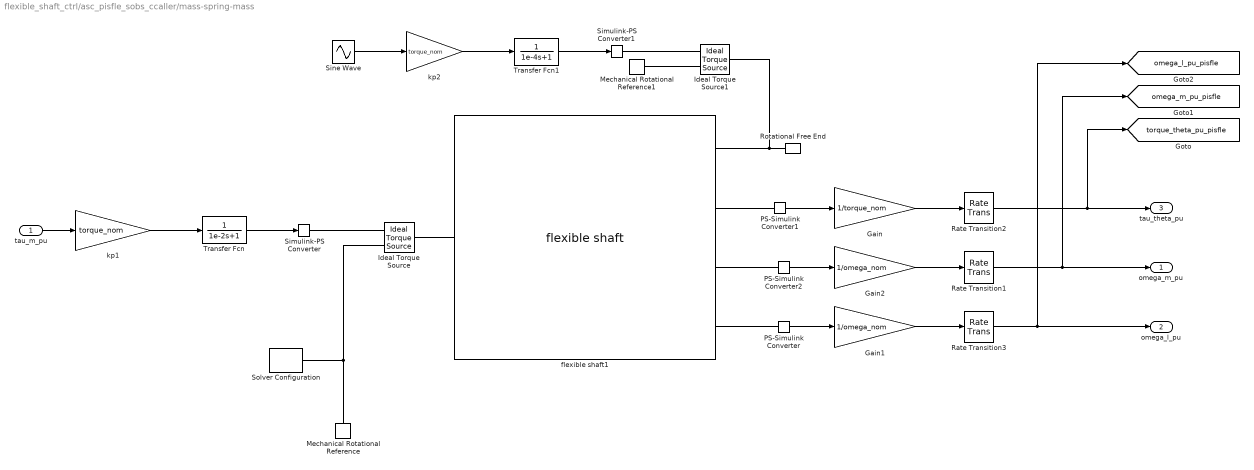
== system flexible_shaft_ctrl/asc_pisfle_sobs_ccaller/mass-spring-mass ==
  tau_m_pu : Inport
  Gain : Gain  Gain=1/torque_nom
  Gain1 : Gain  Gain=1/omega_nom
  Gain2 : Gain  Gain=1/omega_nom
  Ideal Torque Source : fl_lib/Mechanical/Mechanical Sources/Ideal Torque Source
  Ideal Torque Source1 : fl_lib/Mechanical/Mechanical Sources/Ideal Torque Source
  Mechanical Rotational Reference : fl_lib/Mechanical/Rotational Elements/Mechanical Rotational Reference
  Mechanical Rotational Reference1 : fl_lib/Mechanical/Rotational Elements/Mechanical Rotational Reference
  PS-Simulink Converter : nesl_utility/PS-Simulink Converter  PhysicalDomain=network_engine_domain  SubClassName=ps_output  LeftPortType=input  RightPortType=output  PseudoPeriodic=off  Frequencies=[]  VectorFormat=1-D array  Unit=rad/s  AffineConversion=off
  PS-Simulink Converter1 : nesl_utility/PS-Simulink Converter  PhysicalDomain=network_engine_domain  SubClassName=ps_output  LeftPortType=input  RightPortType=output  PseudoPeriodic=off  Frequencies=[]  VectorFormat=1-D array  Unit=N*m  AffineConversion=off
  PS-Simulink Converter2 : nesl_utility/PS-Simulink Converter  PhysicalDomain=network_engine_domain  SubClassName=ps_output  LeftPortType=input  RightPortType=output  PseudoPeriodic=off  Frequencies=[]  VectorFormat=1-D array  Unit=rad/s  AffineConversion=off
  Rate Transition1 : RateTransition  OutPortSampleTime=ts_slow
  Rate Transition2 : RateTransition  OutPortSampleTime=ts_slow
  Rate Transition3 : RateTransition  OutPortSampleTime=ts_slow
  Rotational Free End : fl_lib/Mechanical/Rotational Elements/Rotational Free End  w_specify=off  w_priority=None  w=0 rad/s  w_nominal_specify=off  w_nominal_value=1  w_nominal_unit=rad/s
  Simulink-PS Converter : nesl_utility/Simulink-PS Converter  PhysicalDomain=network_engine_domain  SubClassName=ps_input  LeftPortType=input  RightPortType=output  PseudoPeriodic=off  Frequencies=[]  NoiseDistribution=none  NoiseParameters=[]  Unit=N*m  AffineConversion=off  FilteringAndDerivatives=provide  SimscapeFilterOrder=1  InputFilterTimeConstant=0.001  UdotUserProvided=0
  Simulink-PS Converter1 : nesl_utility/Simulink-PS Converter  PhysicalDomain=network_engine_domain  SubClassName=ps_input  LeftPortType=input  RightPortType=output  PseudoPeriodic=off  Frequencies=[]  NoiseDistribution=none  NoiseParameters=[]  Unit=N*m  AffineConversion=off  FilteringAndDerivatives=provide  SimscapeFilterOrder=1  InputFilterTimeConstant=0.001  UdotUserProvided=0
  Sine Wave : Sin  Amplitude=torque_disturbance  Frequency=f0_min*2*pi  SampleTime=0
  Solver Configuration : nesl_utility/Solver Configuration  PhysicalDomain=network_engine_domain  SubClassName=solver  LeftPortType=input  RightPortType=generic  Tones=[]  Harmonics=[]  SimulateNoise=off  Profile=off  UseLocalSampling=off  EnableSwitchedLinearOptims=on  FrequencyDomain=off  UseCCode=off  RelTol=0.001  AbsTol=0.001  MinStep=1e-09  ToWorkspace=off  RevertToSquareIcSolve=off  NumHomotopyIterations=100  PhasorMode=off  PhasorModeNumHarmonics=1  ConsistencySolver=NEWTON_XTOL_AFTER_FTOL  IndexReductionMethod=DerivativeReplacement  DoDC=off  ResidualTolerance=1e-09  ConsistencyTolSource=GLOBAL  ConsistencyAbsTol=0.001  ConsistencyRelTol=0.001  ConsistencyTolFactor=0.001  UseLocalSolver=on  LocalSolverChoice=NE_BACKWARD_EULER_ADVANCER  ResolveIndetEquations=on  FunctionEvalNumThread=1  LocalSolverSampleTime=tc  DoFixedCost=on  MaxNonlinIter=3  MaxModeIter=2  ComputeImpulses=off  ImpulseIterations=2  LinearAlgebra=auto  LinearAlgebraNumThread=0  EquationFormulation=NE_TIME_EF  DelaysMemoryBudget=1024  AutomaticFiltering=on  FilteringTimeConstant=0.001  PartitionStorageMethod=AS_NEEDED  PartitionMemoryBudget=1024  PartitionMethod=ROBUST  MultibodyUseLocalSolver=off  MultibodyLocalSolverChoice=ODE1  MultibodyLocalSolverSampleTime=0.001
  Transfer Fcn : TransferFcn  Denominator=[1e-2 1]
  Transfer Fcn1 : TransferFcn  Denominator=[1e-4 1]
  flexible shaft1 : flexshaft_2masses_lib/flexible shaft  b1=Dm N*m*s/rad  J1=Jm_model kg*m^2  b2=Dl N*m*s/rad  J2=Jl_model kg*m^2  b_theta=Dtheta N*m*s/rad  k_theta=Ktheta_model N*m/rad  w_1_specify=off  w_1_priority=None  w_1=0 rad/s  w_1_nominal_specify=off  w_1_nominal_value=1  w_1_nominal_unit=rad/s  w_2_specify=off  w_2_priority=None  w_2=0 rad/s  w_2_nominal_specify=off  w_2_nominal_value=1  w_2_nominal_unit=rad/s  t_1_specify=off  t_1_priority=None  t_1=0 N*m  t_1_nominal_specify=off  t_1_nominal_value=1  t_1_nominal_unit=N*m  t_2_specify=off  t_2_priority=None  t_2=0 N*m  t_2_nominal_specify=off  t_2_nominal_value=1  t_2_nominal_unit=N*m  t_theta_specify=off  t_theta_priority=None  t_theta=0 N*m  t_theta_nominal_specify=off  t_theta_nominal_value=1  t_theta_nominal_unit=N*m
      settings: InternalSimscapePortConfiguration="{\"Bottom\":[],\"Left\":[{\"id\":\"S1\",\"label\":\"S1\",\"type\":\"foundation.mechanical.rotational.rotational\"}],\"Right\":[{\"id\":\"S2\",\"label\":\"S2\",\"type\":\"foundation.mechanical.rotational.rotational\"},{\"id\":\"tau_theta\",\"label\":\"tau_theta\",\"type\":\"output\"},{\"id\":\"w1\",\"label\":\"w1\",\"type\":\"output\"},{\"id\":\"w2\",\"label\":\"w2\",\"type\":\"output\"}],\"Top\":[]}"
  kp1 : Gain  Gain=torque_nom  SaturateOnIntegerOverflow=on  OutDataTypeStr=Inherit: Same as input  ParamDataTypeStr=Inherit: Same as input
  kp2 : Gain  Gain=torque_nom  SaturateOnIntegerOverflow=on  OutDataTypeStr=Inherit: Same as input  ParamDataTypeStr=Inherit: Same as input
  omega_m_pu : Outport
  omega_l_pu : Outport  Port=2
  tau_theta_pu : Outport  Port=3
  tag scope: omega_l_pu_pisfle=global, omega_m_pu_pisfle=global, torque_theta_pu_pisfle=global
  wires:
  Sine Wave/1 -> kp2/1
  kp2/1 -> Transfer Fcn1/1
  Transfer Fcn1/1 -> Simulink-PS Converter1/1
  tau_m_pu/1 -> kp1/1
  PS-Simulink Converter2/1 -> Gain2/1
  PS-Simulink Converter/1 -> Gain1/1
  PS-Simulink Converter1/1 -> Gain/1
  Transfer Fcn/1 -> Simulink-PS Converter/1
  kp1/1 -> Transfer Fcn/1
  Gain/1 -> Rate Transition2/1
  Gain2/1 -> Rate Transition1/1
  Gain1/1 -> Rate Transition3/1
  Rate Transition3/1 -> [omega_l_pu_pisfle], omega_l_pu/1
  Rate Transition2/1 -> [torque_theta_pu_pisfle], tau_theta_pu/1
  Rate Transition1/1 -> omega_m_pu/1, [omega_m_pu_pisfle]
  connections:
  Simulink-PS Converter1/RConn1 -- Ideal Torque Source1/RConn1
  Mechanical Rotational Reference1/LConn1 -- Ideal Torque Source1/RConn2
  Ideal Torque Source1/LConn1 -- flexible shaft1/RConn1 -- Rotational Free End/LConn1
  Ideal Torque Source/RConn1 -- Simulink-PS Converter/RConn1
  flexible shaft1/LConn1 -- Ideal Torque Source/LConn1
  Mechanical Rotational Reference/LConn1 -- Solver Configuration/RConn1 -- Ideal Torque Source/RConn2
  flexible shaft1/RConn4 -- PS-Simulink Converter/LConn1
  flexible shaft1/RConn2 -- PS-Simulink Converter1/LConn1
  flexible shaft1/RConn3 -- PS-Simulink Converter2/LConn1
